simulink library "casper_library_misc"  (R2021a)
settings: Solver=ode45  StartTime=0.0  StopTime=10.0  RelTol=1e-3
libraries: xbsIndex_r4 x168, $bdroot x11, xps_library x6, simulink x4
(part 3 of 3)

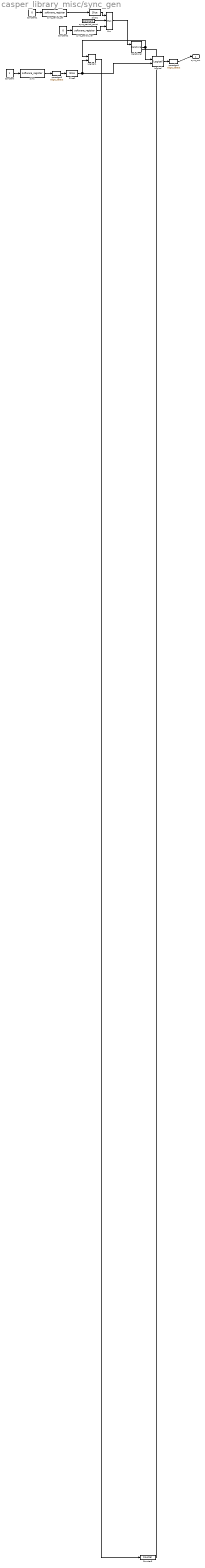
== system casper_library_misc/sync_gen ==
  Constant : Constant
  Constant1 : Constant  Value=0
  Constant2 : Constant  Value=0
  Counter3 : xbsIndex_r4/Counter  cnt_type=Free Running  cnt_to=Inf  operation=Up  start_count=0  cnt_by_val=1  arith_type=Unsigned  n_bits=32  bin_pt=0  load_pin=off  rst=on  en=off  explicit_period=off  period=1  use_behavioral_HDL=off  implementation=Fabric  use_rpm=on  dbl_ovrd=off  block_type=counter
      settings: xl_area=[0, 0, 0, 0, 0, 0, 0]
  Logical : xbsIndex_r4/Logical  logical_function=OR  inputs=2  en=off  latency=0  precision=Full  arith_type=Unsigned  n_bits=8  bin_pt=2  align_bp=on  dbl_ovrd=off  block_type=logical
      settings: xl_area=[0, 0, 0, 0, 0, 0, 0]
  Logical1 : xbsIndex_r4/Logical  logical_function=OR  inputs=2  en=off  latency=0  precision=Full  arith_type=Unsigned  n_bits=8  bin_pt=2  align_bp=on  dbl_ovrd=off  block_type=logical
      settings: xl_area=[0, 0, 0, 0, 0, 0, 0]
  Mux : xbsIndex_r4/Mux  inputs=2  en=off  latency=0  precision=Full  arith_type=Unsigned  n_bits=16  bin_pt=14  quantization=Truncate  overflow=Wrap  dbl_ovrd=off  block_type=mux
  Relational : xbsIndex_r4/Relational  mode=a=b  op_type=Bool  en=off  latency=1  dbl_ovrd=off  block_type=relational
      settings: xl_area=[0, 0, 0, 0, 0, 0, 0]  block_version=10.1.3
  Slice1 : xbsIndex_r4/Slice  nbits=1  boolean_output=on  mode=Lower Bit Location + Width  bit1=0  base1=MSB of Input  bit0=0  base0=LSB of Input  dbl_ovrd=off  block_type=slice
      settings: infoedit="Extracts a given range of bits from each input sample and presents it at the output.  The output type is ordinarily unsigned with binary point at zero, but can be Boolean when the slice is one bit wide.<P><P>Hardware notes: In hardware this block costs nothing."  block_version=10.1.3
  Slice2 : xbsIndex_r4/Slice  nbits=1  boolean_output=on  mode=Lower Bit Location + Width  bit1=0  base1=MSB of Input  bit0=0  base0=LSB of Input  dbl_ovrd=off  block_type=slice
      settings: infoedit="Extracts a given range of bits from each input sample and presents it at the output.  The output type is ordinarily unsigned with binary point at zero, but can be Boolean when the slice is one bit wide.<P><P>Hardware notes: In hardware this block costs nothing."  block_version=10.1.3
  posedge1 : $bdroot/edge_detect  edge=Rising  polarity=Active High  x_in=[0 0.08 0.08 0.16 0.16 0.24 0.24 0.32 0.32 0.4]  y_in="[-1 -1  1  1  1  1  1  1  1  1]"  x_out=[0.6 0.68 0.68 0.76 0.76 0.84 0.84 0.92 0.92 1]  y_out="[-1 -1  1  1 -1 -1 -1 -1 -1 -1]"
      settings: AttributesFormatString=|
      | rising edges
      | active high
  posedge3 : $bdroot/edge_detect  edge=Rising  polarity=Active High  x_in=[0 0.08 0.08 0.16 0.16 0.24 0.24 0.32 0.32 0.4]  y_in="[-1 -1  1  1  1  1  1  1  1  1]"  x_out=[0.6 0.68 0.68 0.76 0.76 0.84 0.84 0.92 0.92 1]  y_out="[-1 -1  1  1 -1 -1 -1 -1 -1 -1]"
      settings: AttributesFormatString=|
      | rising edges
      | active high
  sync : xps_library/Memory/software_register  Tag=xps:sw_reg  io_dir=From Processor  io_delay=0  init_val=0  sample_period=1  names=reg  bitwidths=32  bin_pts=0  arith_types=0  sim_port=on  show_format=on
      settings: AttributesFormatString=1input:uf32.0 = 32 bits  SourceProductName=CASPER XPS Blockset
  sync_period_const : xbsIndex_r4/Constant  const=8958  gui_display_data_type=Fixed-point  arith_type=Signed (2's comp)  n_bits=32  bin_pt=0  preci_type=Single  exp_width=8  frac_width=24  explicit_period=off  period=1  equ=P=C  opselect=C  inp2=PCIN>>17  opr=+  inp1=P  carry=CIN  dbl_ovrd=off  block_type=constant
      settings: block_version=10.1.1
  sync_period_sel : xps_library/Memory/software_register  Tag=xps:sw_reg  io_dir=From Processor  io_delay=0  init_val=0  sample_period=1  names=reg  bitwidths=32  bin_pts=0  arith_types=0  sim_port=on  show_format=on
      settings: AttributesFormatString=1input:uf32.0 = 32 bits  SourceProductName=CASPER XPS Blockset
  sync_period_var : xps_library/Memory/software_register  Tag=xps:sw_reg  io_dir=From Processor  io_delay=0  init_val=0  sample_period=1  names=reg  bitwidths=32  bin_pts=0  arith_types=0  sim_port=on  show_format=on
      settings: AttributesFormatString=1input:uf32.0 = 32 bits  SourceProductName=CASPER XPS Blockset
  sync_out : Outport  VectorParamsAs1DForOutWhenUnconnected=off
  wires:
  posedge3/1 -> Slice2/1
  Slice2/1 -> Logical1/2, Logical/2
  Logical1/1 -> Counter3/1
  Counter3/1 -> Relational/2
  Relational/1 -> Logical/1, Logical1/1
  Logical/1 -> posedge1/1
  posedge1/1 -> sync_out/1
  Mux/1 -> Relational/1
  Slice1/1 -> Mux/1
  sync_period_const/1 -> Mux/2
  Constant1/1 -> sync_period_sel/1
  Constant2/1 -> sync_period_var/1
  Constant/1 -> sync/1
  sync_period_var/1 -> Mux/3
  sync_period_sel/1 -> Slice1/1
  sync/1 -> posedge3/1

== system casper_library_misc/test ==

== system casper_library_misc/triggered_counter ==
  trig : Inport
  Counter : xbsIndex_r4/Counter  cnt_type=Free Running  cnt_to=Inf  operation=Up  start_count=2^(nextpow2(len)+1)-len  cnt_by_val=1  arith_type=Unsigned  n_bits=nextpow2(len)+1  bin_pt=0  load_pin=off  rst=on  en=on  explicit_period=on  period=1  use_behavioral_HDL=off  implementation=Fabric  use_rpm=on  dbl_ovrd=off  block_type=counter
      settings: xl_area=[0, 0, 0, 0, 0, 0, 0]
  all_but_msb : xbsIndex_r4/Slice  nbits=1  boolean_output=off  mode=Two Bit Locations  bit1=-1  base1=MSB of Input  bit0=0  base0=LSB of Input  dbl_ovrd=off  block_type=slice
      settings: infoedit="Extracts a given range of bits from each input sample and presents it at the output.  The output type is ordinarily unsigned with binary point at zero, but can be Boolean when the slice is one bit wide.<P><P>Hardware notes: In hardware this block costs nothing."  block_version=10.1.3
  edge_detect : Subsystem  mask(edge_detect){edge=Rising, polarity=Active High, xin=floor([0.5:0.5:5])*0.08, yin={[-1,-1,1,1,1,1,1,1,1,1],[1,1,-1,-1,-1,-1,-1,-1,-1,-1],[-1,-1,1,1,1,1,-1,-1,-1,-1]}, xout=1-floor([5:-0.5:0.5])*0.08, yout={[-1,-1,1,1,-1,-1,-1,-1,-1,-1],[-1,-1,1,1,-1,-1,-1,-1,-1,-1],[-1,-1,1,1,-1,-1,1,1,-1,-1]}}
      mask prompts: edge "Edge Type"; polarity "Output Polarity"; xin "Input X Positions"; yin "Input Y Positions"; xout "Output X Positions"; yout "Output Y Positions"
      mask help: Output is active for one-cycle after each edge of the specified type (i.e. rising, falling or both).
      mask init:
      | edge_detect_init(gcb,edge,polarity);
      settings: AttributesFormatString=|
      | rising edges
      | active high
      mask Help: Output is active for one-cycle after each edge of the specified type (i.e. rising, falling, or both).  Latency is zero.
      mask TypeOptions edge: Rising | Falling | Both
      mask TypeOptions polarity: Active High | Active Low
      mask Display:
      | plot(xin,0.5+yin{edge}*0.2)
      | plot(xout,0.5+yout{edge}*0.2*(3-2*polarity))
  msb : xbsIndex_r4/Slice  nbits=1  boolean_output=on  mode=Upper Bit Location + Width  bit1=0  base1=MSB of Input  bit0=0  base0=LSB of Input  dbl_ovrd=off  block_type=slice
      settings: infoedit="Extracts a given range of bits from each input sample and presents it at the output.  The output type is ordinarily unsigned with binary point at zero, but can be Boolean when the slice is one bit wide.<P><P>Hardware notes: In hardware this block costs nothing."  block_version=10.1.3
  count : Outport  VectorParamsAs1DForOutWhenUnconnected=off
  valid : Outport  Port=2  VectorParamsAs1DForOutWhenUnconnected=off
  wires:
  trig/1 -> edge_detect/1(in)
  msb/1 -> Counter/2, valid/1
  Counter/1 -> msb/1, all_but_msb/1
  edge_detect/1(out) -> Counter/1
  all_but_msb/1 -> count/1

== system casper_library_misc/armed_trigger/edge_detect ==
  in : Inport
  Delay : xbsIndex_r4/Delay  rst=off  infoeditControl=Selection of Reset will increase slice count due to use of real FFs and instead of SRLs  en=off  latency=1  reg_retiming=off  dbl_ovrd=off  block_type=delay
      settings: xl_area=[0, 0, 0, 0, 0, 0, 0]
  Inverter : xbsIndex_r4/Inverter  en=off  latency=0  dbl_ovrd=off  block_type=inv
      settings: xl_area=[0, 0, 0, 0, 0, 0, 0]
  edge_op : xbsIndex_r4/Logical  logical_function=NOR  inputs=2  en=off  latency=0  precision=Full  arith_type=Unsigned  n_bits=8  bin_pt=2  align_bp=on  dbl_ovrd=off  block_type=logical
      settings: xl_area=[0, 0, 0, 0, 0, 0, 0]
  out : Outport  VectorParamsAs1DForOutWhenUnconnected=off
  wires:
  Inverter/1 -> edge_op/1
  edge_op/1 -> out/1
  in/1 -> Inverter/1, Delay/1
  Delay/1 -> edge_op/2

== system casper_library_misc/fixed_to_float/debus ==
  bus_in : Inport
  reinterpret1 : xbsIndex_r4/Reinterpret  force_arith_type=on  arith_type="Signed  (2's comp)"  force_bin_pt=on  bin_pt=17  block_type=reinterpret
  slice1 : xbsIndex_r4/Slice  nbits=18  boolean_output=off  mode=Upper Bit Location + Width  bit1=0  base1=MSB of Input  bit0=0  base0=LSB of Input  dbl_ovrd=off  block_type=slice
  msb_lsb_out1 : Outport
  wires:
  bus_in/1 -> slice1/1
  slice1/1 -> reinterpret1/1
  reinterpret1/1 -> msb_lsb_out1/1

== system casper_library_misc/triggered_counter/edge_detect ==
  in : Inport
  Delay : xbsIndex_r4/Delay  rst=off  infoeditControl=Selection of Reset will increase slice count due to use of real FFs and instead of SRLs  en=off  latency=1  reg_retiming=off  dbl_ovrd=off  block_type=delay
      settings: xl_area=[0, 0, 0, 0, 0, 0, 0]
  Inverter : xbsIndex_r4/Inverter  en=off  latency=0  dbl_ovrd=off  block_type=inv
      settings: xl_area=[0, 0, 0, 0, 0, 0, 0]
  edge_op : xbsIndex_r4/Logical  logical_function=NOR  inputs=2  en=off  latency=0  precision=Full  arith_type=Unsigned  n_bits=8  bin_pt=2  align_bp=on  dbl_ovrd=off  block_type=logical
      settings: xl_area=[0, 0, 0, 0, 0, 0, 0]
  out : Outport  VectorParamsAs1DForOutWhenUnconnected=off
  wires:
  Inverter/1 -> edge_op/1
  edge_op/1 -> out/1
  in/1 -> Inverter/1, Delay/1
  Delay/1 -> edge_op/2
